simulink model "Simulink_1_Motor_Sin_Control"  (R2025b)
settings: Solver=ode45  StartTime=0.0  StopTime=2.5  MaxStep=0.005  RelTol=1e-3
settings Model: Creator=juanj  LastModifiedBy=juanj

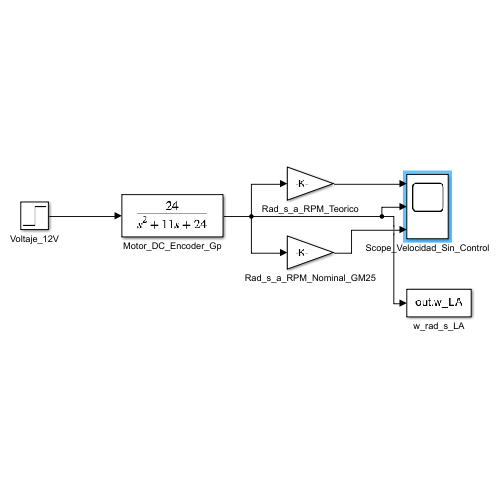
[thumbnail: Simulink's stored preview of the top-level diagram]
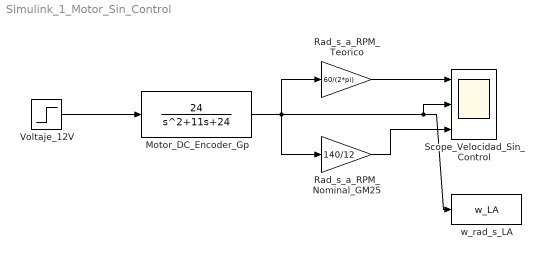
== system Simulink_1_Motor_Sin_Control ==
  Motor_DC_Encoder_Gp : TransferFcn  Numerator=[24]  Denominator=[1 11 24]
  Rad_s_a_RPM_Nominal_GM25 : Gain  Gain=140/12
  Rad_s_a_RPM_Teorico : Gain  Gain=60/(2*pi)
  Scope_Velocidad_Sin_Control : Scope  NumInputPorts=3
      settings: ActiveDisplayYMinimum=-17.484513659277944  ActiveDisplayYMaximum=157.36062293350153
  Voltaje_12V : Step  Time=0  After=12  SampleTime=0
  w_rad_s_LA : ToWorkspace  VariableName=w_LA  SaveFormat=Timeseries  SampleTime=-1
  wires:
  Voltaje_12V/1 -> Motor_DC_Encoder_Gp/1
  Motor_DC_Encoder_Gp/1 -> Scope_Velocidad_Sin_Control/2, w_rad_s_LA/1, Rad_s_a_RPM_Teorico/1, Rad_s_a_RPM_Nominal_GM25/1
  Rad_s_a_RPM_Teorico/1 -> Scope_Velocidad_Sin_Control/1
  Rad_s_a_RPM_Nominal_GM25/1 -> Scope_Velocidad_Sin_Control/3
